simulink model "spherical_wrist"  (R2023b)
settings: Solver=VariableStepAuto  StartTime=0.0  StopTime=20  FixedStep=0.001  RelTol=1e-3
InitFcn:
  | WRIST_60_50_DataFile
model workspace (MAT data in the model file):
  Damp : Simulink.Parameter (value not decoded)
  Dm : Simulink.Parameter (value not decoded)
  Jm : Simulink.Parameter (value not decoded)
  Km : Simulink.Parameter (value not decoded)
  Tc : Simulink.Parameter (value not decoded)
values from neighbouring files (symbols this model uses):
  PQ = [P(1,:)*Q(1,:)' P(2,:)*Q(2,:)' P(3,:)*Q(3,:)']    [WRIST_60_50_DataFile.m]
  Pz = -tand(30)*[1; 1; 1]    [WRIST_60_50_DataFile.m]
  Q = [cosd(plat_off) sind(plat_off) [0; 0; 0]]    [WRIST_60_50_DataFile.m]
symbols that are objects in the model workspace (value not decoded): Damp, Dm, Tc
undefined symbols (not defined in the file or in its folder): smiData, X, Y, Z
libraries: sm_lib x44, nesl_utility x20, fl_lib x15, sdl_lib x9, sharedtransform x2, slpidlib x1
(part 3 of 3)

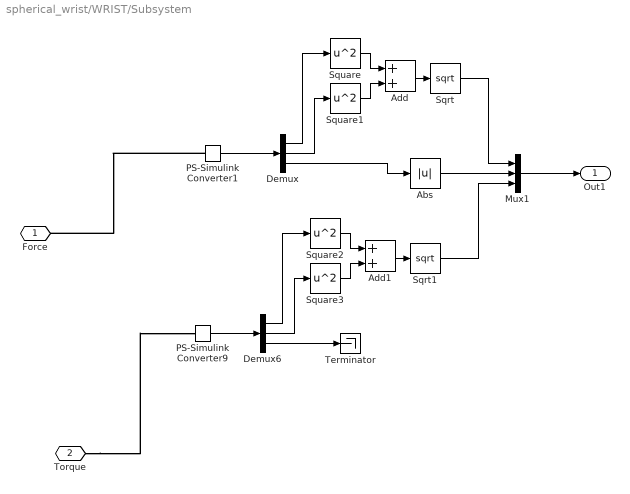
== system spherical_wrist/WRIST/Subsystem ==
  Abs : Abs  SaturateOnIntegerOverflow=off
  Add : Sum
  Add1 : Sum
  Demux : Demux  Outputs=3
  Demux6 : Demux  Outputs=3
  Mux1 : Mux  Inputs=3
  PS-Simulink Converter1 : nesl_utility/PS-Simulink Converter  PhysicalDomain=network_engine_domain  SubClassName=ps_output  LeftPortType=input  RightPortType=output  PseudoPeriodic=off  Frequencies=[]  VectorFormat=1-D array  Unit=N  AffineConversion=off
  PS-Simulink Converter9 : nesl_utility/PS-Simulink Converter  PhysicalDomain=network_engine_domain  SubClassName=ps_output  LeftPortType=input  RightPortType=output  PseudoPeriodic=off  Frequencies=[]  VectorFormat=1-D array  Unit=N*m  AffineConversion=off
  Sqrt : Sqrt
  Sqrt1 : Sqrt
  Square{,1..3} (4 alike) : Math  Operator=square
  Terminator : Terminator
  Force : PMIOPort  Side=Left
  Torque : PMIOPort  Port=2  Side=Left
  Out1 : Outport
  wires:
  Add1/1 -> Sqrt1/1
  Demux/2 -> Square1/1
  Demux/3 -> Abs/1
  Demux6/1 -> Square2/1
  PS-Simulink Converter1/1 -> Demux/1
  Square/1 -> Add/1
  Add/1 -> Sqrt/1
  PS-Simulink Converter9/1 -> Demux6/1
  Demux6/3 -> Terminator/1
  Sqrt1/1 -> Mux1/3
  Sqrt/1 -> Mux1/1
  Square1/1 -> Add/2
  Demux/1 -> Square/1
  Demux6/2 -> Square3/1
  Square2/1 -> Add1/1
  Square3/1 -> Add1/2
  Mux1/1 -> Out1/1
  Abs/1 -> Mux1/2
  connections:
  PS-Simulink Converter1/LConn1 -- Force/RConn1
  Torque/RConn1 -- PS-Simulink Converter9/LConn1

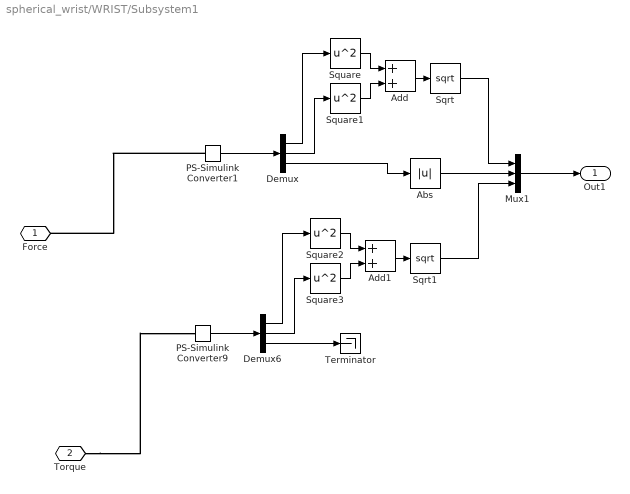
== system spherical_wrist/WRIST/Subsystem1 ==
  Abs : Abs  SaturateOnIntegerOverflow=off
  Add : Sum
  Add1 : Sum
  Demux : Demux  Outputs=3
  Demux6 : Demux  Outputs=3
  Mux1 : Mux  Inputs=3
  PS-Simulink Converter1 : nesl_utility/PS-Simulink Converter  PhysicalDomain=network_engine_domain  SubClassName=ps_output  LeftPortType=input  RightPortType=output  PseudoPeriodic=off  Frequencies=[]  VectorFormat=1-D array  Unit=N  AffineConversion=off
  PS-Simulink Converter9 : nesl_utility/PS-Simulink Converter  PhysicalDomain=network_engine_domain  SubClassName=ps_output  LeftPortType=input  RightPortType=output  PseudoPeriodic=off  Frequencies=[]  VectorFormat=1-D array  Unit=N*m  AffineConversion=off
  Sqrt : Sqrt
  Sqrt1 : Sqrt
  Square{,1..3} (4 alike) : Math  Operator=square
  Terminator : Terminator
  Force : PMIOPort  Side=Left
  Torque : PMIOPort  Port=2  Side=Left
  Out1 : Outport
  wires:
  Add1/1 -> Sqrt1/1
  Demux/2 -> Square1/1
  Demux/3 -> Abs/1
  Demux6/1 -> Square2/1
  PS-Simulink Converter1/1 -> Demux/1
  Square/1 -> Add/1
  Add/1 -> Sqrt/1
  PS-Simulink Converter9/1 -> Demux6/1
  Demux6/3 -> Terminator/1
  Sqrt1/1 -> Mux1/3
  Sqrt/1 -> Mux1/1
  Square1/1 -> Add/2
  Demux/1 -> Square/1
  Demux6/2 -> Square3/1
  Square2/1 -> Add1/1
  Square3/1 -> Add1/2
  Mux1/1 -> Out1/1
  Abs/1 -> Mux1/2
  connections:
  PS-Simulink Converter1/LConn1 -- Force/RConn1
  Torque/RConn1 -- PS-Simulink Converter9/LConn1

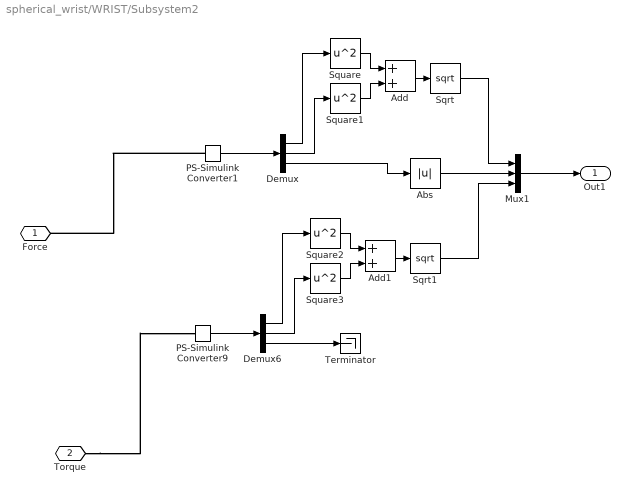
== system spherical_wrist/WRIST/Subsystem2 ==
  Abs : Abs  SaturateOnIntegerOverflow=off
  Add : Sum
  Add1 : Sum
  Demux : Demux  Outputs=3
  Demux6 : Demux  Outputs=3
  Mux1 : Mux  Inputs=3
  PS-Simulink Converter1 : nesl_utility/PS-Simulink Converter  PhysicalDomain=network_engine_domain  SubClassName=ps_output  LeftPortType=input  RightPortType=output  PseudoPeriodic=off  Frequencies=[]  VectorFormat=1-D array  Unit=N  AffineConversion=off
  PS-Simulink Converter9 : nesl_utility/PS-Simulink Converter  PhysicalDomain=network_engine_domain  SubClassName=ps_output  LeftPortType=input  RightPortType=output  PseudoPeriodic=off  Frequencies=[]  VectorFormat=1-D array  Unit=N*m  AffineConversion=off
  Sqrt : Sqrt
  Sqrt1 : Sqrt
  Square{,1..3} (4 alike) : Math  Operator=square
  Terminator : Terminator
  Force : PMIOPort  Side=Left
  Torque : PMIOPort  Port=2  Side=Left
  Out1 : Outport
  wires:
  Add1/1 -> Sqrt1/1
  Demux/2 -> Square1/1
  Demux/3 -> Abs/1
  Demux6/1 -> Square2/1
  PS-Simulink Converter1/1 -> Demux/1
  Square/1 -> Add/1
  Add/1 -> Sqrt/1
  PS-Simulink Converter9/1 -> Demux6/1
  Demux6/3 -> Terminator/1
  Sqrt1/1 -> Mux1/3
  Sqrt/1 -> Mux1/1
  Square1/1 -> Add/2
  Demux/1 -> Square/1
  Demux6/2 -> Square3/1
  Square2/1 -> Add1/1
  Square3/1 -> Add1/2
  Mux1/1 -> Out1/1
  Abs/1 -> Mux1/2
  connections:
  PS-Simulink Converter1/LConn1 -- Force/RConn1
  Torque/RConn1 -- PS-Simulink Converter9/LConn1

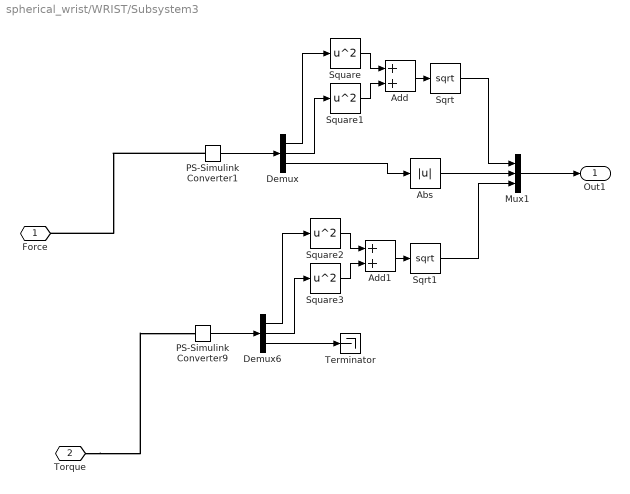
== system spherical_wrist/WRIST/Subsystem3 ==
  Abs : Abs  SaturateOnIntegerOverflow=off
  Add : Sum
  Add1 : Sum
  Demux : Demux  Outputs=3
  Demux6 : Demux  Outputs=3
  Mux1 : Mux  Inputs=3
  PS-Simulink Converter1 : nesl_utility/PS-Simulink Converter  PhysicalDomain=network_engine_domain  SubClassName=ps_output  LeftPortType=input  RightPortType=output  PseudoPeriodic=off  Frequencies=[]  VectorFormat=1-D array  Unit=N  AffineConversion=off
  PS-Simulink Converter9 : nesl_utility/PS-Simulink Converter  PhysicalDomain=network_engine_domain  SubClassName=ps_output  LeftPortType=input  RightPortType=output  PseudoPeriodic=off  Frequencies=[]  VectorFormat=1-D array  Unit=N*m  AffineConversion=off
  Sqrt : Sqrt
  Sqrt1 : Sqrt
  Square{,1..3} (4 alike) : Math  Operator=square
  Terminator : Terminator
  Force : PMIOPort  Side=Left
  Torque : PMIOPort  Port=2  Side=Left
  Out1 : Outport
  wires:
  Add1/1 -> Sqrt1/1
  Demux/2 -> Square1/1
  Demux/3 -> Abs/1
  Demux6/1 -> Square2/1
  PS-Simulink Converter1/1 -> Demux/1
  Square/1 -> Add/1
  Add/1 -> Sqrt/1
  PS-Simulink Converter9/1 -> Demux6/1
  Demux6/3 -> Terminator/1
  Sqrt1/1 -> Mux1/3
  Sqrt/1 -> Mux1/1
  Square1/1 -> Add/2
  Demux/1 -> Square/1
  Demux6/2 -> Square3/1
  Square2/1 -> Add1/1
  Square3/1 -> Add1/2
  Mux1/1 -> Out1/1
  Abs/1 -> Mux1/2
  connections:
  PS-Simulink Converter1/LConn1 -- Force/RConn1
  Torque/RConn1 -- PS-Simulink Converter9/LConn1

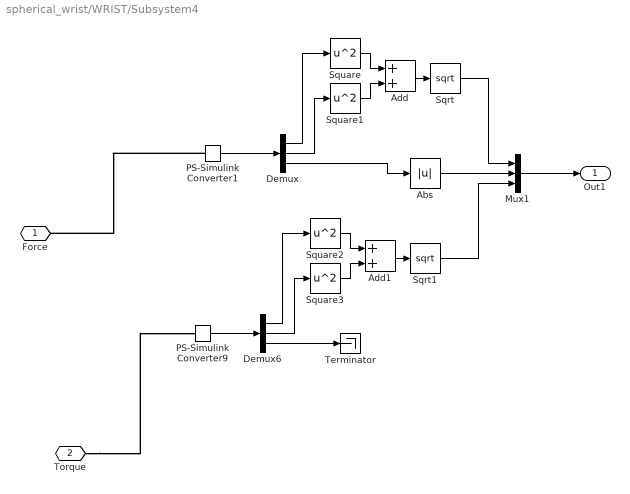
== system spherical_wrist/WRIST/Subsystem4 ==
  Abs : Abs  SaturateOnIntegerOverflow=off
  Add : Sum
  Add1 : Sum
  Demux : Demux  Outputs=3
  Demux6 : Demux  Outputs=3
  Mux1 : Mux  Inputs=3
  PS-Simulink Converter1 : nesl_utility/PS-Simulink Converter  PhysicalDomain=network_engine_domain  SubClassName=ps_output  LeftPortType=input  RightPortType=output  PseudoPeriodic=off  Frequencies=[]  VectorFormat=1-D array  Unit=N  AffineConversion=off
  PS-Simulink Converter9 : nesl_utility/PS-Simulink Converter  PhysicalDomain=network_engine_domain  SubClassName=ps_output  LeftPortType=input  RightPortType=output  PseudoPeriodic=off  Frequencies=[]  VectorFormat=1-D array  Unit=N*m  AffineConversion=off
  Sqrt : Sqrt
  Sqrt1 : Sqrt
  Square{,1..3} (4 alike) : Math  Operator=square
  Terminator : Terminator
  Force : PMIOPort  Side=Left
  Torque : PMIOPort  Port=2  Side=Left
  Out1 : Outport
  wires:
  Add1/1 -> Sqrt1/1
  Demux/2 -> Square1/1
  Demux/3 -> Abs/1
  Demux6/1 -> Square2/1
  PS-Simulink Converter1/1 -> Demux/1
  Square/1 -> Add/1
  Add/1 -> Sqrt/1
  PS-Simulink Converter9/1 -> Demux6/1
  Demux6/3 -> Terminator/1
  Sqrt1/1 -> Mux1/3
  Sqrt/1 -> Mux1/1
  Square1/1 -> Add/2
  Demux/1 -> Square/1
  Demux6/2 -> Square3/1
  Square2/1 -> Add1/1
  Square3/1 -> Add1/2
  Mux1/1 -> Out1/1
  Abs/1 -> Mux1/2
  connections:
  PS-Simulink Converter1/LConn1 -- Force/RConn1
  Torque/RConn1 -- PS-Simulink Converter9/LConn1

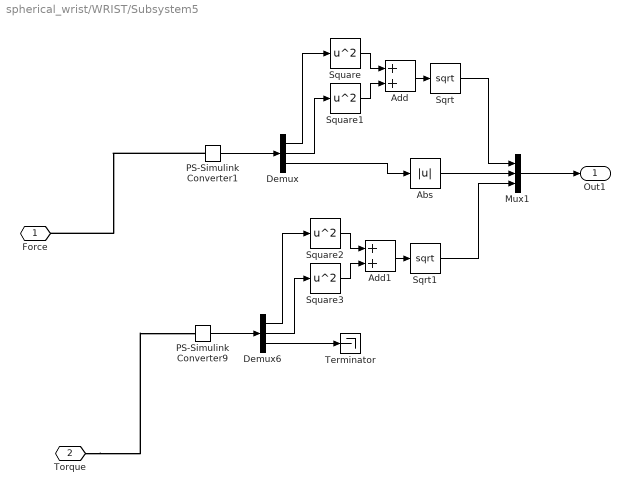
== system spherical_wrist/WRIST/Subsystem5 ==
  Abs : Abs  SaturateOnIntegerOverflow=off
  Add : Sum
  Add1 : Sum
  Demux : Demux  Outputs=3
  Demux6 : Demux  Outputs=3
  Mux1 : Mux  Inputs=3
  PS-Simulink Converter1 : nesl_utility/PS-Simulink Converter  PhysicalDomain=network_engine_domain  SubClassName=ps_output  LeftPortType=input  RightPortType=output  PseudoPeriodic=off  Frequencies=[]  VectorFormat=1-D array  Unit=N  AffineConversion=off
  PS-Simulink Converter9 : nesl_utility/PS-Simulink Converter  PhysicalDomain=network_engine_domain  SubClassName=ps_output  LeftPortType=input  RightPortType=output  PseudoPeriodic=off  Frequencies=[]  VectorFormat=1-D array  Unit=N*m  AffineConversion=off
  Sqrt : Sqrt
  Sqrt1 : Sqrt
  Square{,1..3} (4 alike) : Math  Operator=square
  Terminator : Terminator
  Force : PMIOPort  Side=Left
  Torque : PMIOPort  Port=2  Side=Left
  Out1 : Outport
  wires:
  Add1/1 -> Sqrt1/1
  Demux/2 -> Square1/1
  Demux/3 -> Abs/1
  Demux6/1 -> Square2/1
  PS-Simulink Converter1/1 -> Demux/1
  Square/1 -> Add/1
  Add/1 -> Sqrt/1
  PS-Simulink Converter9/1 -> Demux6/1
  Demux6/3 -> Terminator/1
  Sqrt1/1 -> Mux1/3
  Sqrt/1 -> Mux1/1
  Square1/1 -> Add/2
  Demux/1 -> Square/1
  Demux6/2 -> Square3/1
  Square2/1 -> Add1/1
  Square3/1 -> Add1/2
  Mux1/1 -> Out1/1
  Abs/1 -> Mux1/2
  connections:
  PS-Simulink Converter1/LConn1 -- Force/RConn1
  Torque/RConn1 -- PS-Simulink Converter9/LConn1

== system spherical_wrist/Position_Controller/wrist_decoupler/motors2ypr ==
  theta_meas : Inport
  Gain3 : Gain  Gain=180/pi
  Quaternions to Rotation Angles1 : sharedtransform/Quaternions to Rotation Angles  rotationOrder=ZYX  aMode=aMode
  motors2quat : MATLAB Function  TreatAsAtomicUnit=on
      settings: MinAlgLoopOccurrences=on
  ypr_meas : Outport
  singularity : Outport  Port=2
  cycles : Outport  Port=3
  wires:
  theta_meas/1 -> motors2quat/1(theta_meas)
  Quaternions to Rotation Angles1/1 -> Gain3/1
  Gain3/1 -> ypr_meas/1
  motors2quat/1(attitude) -> Quaternions to Rotation Angles1/1
  motors2quat/2(singularity) -> singularity/1
  motors2quat/3(cycles) -> cycles/1

== matlab function spherical_wrist/Position_Controller/wrapTo180 ==
  data: u input; y output
function y = wrap(u)

y = u;

for k=1:3
    while y(k) > 180.0
        y(k) = y(k) - 360.0;
    end

    while y(k) < -180.0
        y(k) = y(k) + 360.0;
    end
end

== matlab function spherical_wrist/Position_Controller/wrist_decoupler/ypr2motors ==
  data: ypr input; theta output; out_of_range output; PQ parameter; Q parameter; Pz parameter
function [theta,out_of_range] = ypr2motors(ypr, PQ, Q, Pz)

theta = [0;0;0];

q = Q*eul2rotm(deg2rad(ypr'))';
%q = rotatepoint(quaternion(eul2quat(deg2rad([y p r]))),Q);
    
m = [sqrt(q(1,1)^2+q(1,2)^2) sqrt(q(2,1)^2+q(2,2)^2) sqrt(q(3,1)^2+q(3,2)^2)];

if min(abs(m)) == 0
    % out of mechanical motion range
    out_of_range = 1;
    return;
end
    
arg = [(PQ(1)-Pz(1)*q(1,3))/m(1); (PQ(2)-Pz(2)*q(2,3))/m(2); (PQ(3)-Pz(3)*q(3,3))/m(3)];
    
if max(abs(arg)) > 1
    % out of mechanical motion range
    out_of_range = 1;
    return;
end
    
theta = atan2d(q(:,2),q(:,1))+[90; 90; 90;]-asind(arg);
        
out_of_range = 0;

== matlab function spherical_wrist/Position_Controller/wrist_decoupler/motors2ypr/motors2quat ==
  settings: sampleTime=0.1
  data: theta_meas input; attitude output; singularity output; cycles output; Q parameter; PQ parameter; Pz parameter
function [attitude,singularity,cycles] = motors2quat(theta_meas, Q, PQ, Pz)

persistent T;
persistent singularity_reg;

if isempty(T)
    T = quaternion(1,0,0,0);
end

if isempty(singularity_reg)
    singularity_reg = 0;
end

theta_diff = theta_meas - [145; -90; 40];

for k=1:3
    while theta_diff(k) > 180.0
        theta_diff(k) = theta_diff(k) - 360.0;
    end

    while theta_diff(k) < -180.0
        theta_diff(k) = theta_diff(k) + 360.0;
    end
end

%%%%%%%%%%%%%%%%%%%%%%%%%%%%%%%%%%%%%%%%%%%%%%%%%%%%

% if singularity happened, waits for position home
if max(abs(theta_diff)) < 5.0
    singularity_reg = 0;
end

if singularity_reg
    attitude = compact(T);
    singularity = singularity_reg;
    cycles = 0;
    return;
end

%%%%%%%%%%%%%%%%%%%%%%%%%%%%%%%%%%%%%%%%%%%%%%%%%%%%

for cycles=1:200
    
    q = rotatepoint(T,Q);
    
    %%%%%%%%%%%%%%%%%%%%%%%%%%%%%%%%%%%%%%%%%%%%%%%%%%%%%%%%%%%%%%%%%%%%%%%
    
    m = [sqrt(q(1,1)^2+q(1,2)^2) sqrt(q(2,1)^2+q(2,2)^2) sqrt(q(3,1)^2+q(3,2)^2)];

    if min(abs(m)) == 0
        % out of mechanical motion range
        cycles = -1;
        break;
    end
    
    arg = [(PQ(1)-Pz(1)*q(1,3))/m(1); (PQ(2)-Pz(2)*q(2,3))/m(2); (PQ(3)-Pz(3)*q(3,3))/m(3)];
    
    if max(abs(arg)) > 1.0
        % out of mechanical motion range
        cycles = -2;
        break;
    end
    
    theta = atan2d(q(:,2),q(:,1))+[90; 90; 90;]-asind(arg);
    
    %%%%%%%%%%%%%%%%%%%%%%%%%%%%%%%%%%%%%%%%%%%%%%%%%%%%%%%%%%%%%%%%%%%%%%%
    
    theta_err = theta_meas-theta;
    
    for k=1:3
        while theta_err(k) > 180.0
            theta_err(k) = theta_err(k) - 360.0;
        end

        while theta_err(k) < -180.0
            theta_err(k) = theta_err(k) + 360.0;
        end
    end
        
    if max(abs(theta_err)) < 0.01
        T = normalize(T);
        attitude = compact(T);
        singularity = singularity_reg;
        return;
    end
        
    p = [cosd(theta) sind(theta) Pz];
        
    q1xp1 = cross(q(1,:),p(1,:));
    q2xp2 = cross(q(2,:),p(2,:));
    q3xp3 = cross(q(3,:),p(3,:));
        
    if min(abs([q1xp1(3) q2xp2(3) q3xp3(3)])) == 0.0
        % ill jacobian
        cycles = -3;
        break;
    end
        
    if det([q1xp1/q1xp1(3); q2xp2/q2xp2(3); q3xp3/q3xp3(3)]) == 0.0
        % ill jacobian
        cycles = -4;
        break;
    end
        
    T = quaternion(([q1xp1/q1xp1(3); q2xp2/q2xp2(3); q3xp3/q3xp3(3)]\(0.02*theta_err))','rotvec')*T;
end

T = quaternion(1,0,0,0);
attitude = compact(T);
singularity_reg = 1;
singularity = singularity_reg;
